simulink model "Grid_Following_Inverters"  (R2024b)
settings: Solver=VariableStepAuto  StartTime=0.0  StopTime=1  RelTol=1e-3
InitFcn:
  | addpath(genpath(fullfile(fileparts(fileparts(fileparts(get_param(bdroot,'FileName')))),'code','functions')));initialize_equipment_model_from_callback(bdroot);
undefined symbols (not defined in the file): Cf, CL, Delta_Iq_LVRT_max, f, I_base, I_limit, I_N, Id_ref_manual, Iq_ref_manual, K_q_LVRT, L1, L2, Lg, Manual_Current_Ref, PLL, PQ, R_C, R_L1, R_L2, Rg, V_base_phase, V_in, V_LVRT_max, V_LVRT_min, Vg
libraries: spsabctodq0Lib x4, spsControlledVoltageSourceLib x3, spsCurrentMeasurementLib x3, spsThreePhaseSeriesRLCBranchLib x3, spsVoltageMeasurementLib x3, spsThreePhaseVIMeasurementLib x2, slpidlib x2, spsGroundLib x1, spsPLL3phLib x1, spsdq0toabcLib x1, spsThreePhaseBreakerLib x1, spsThreePhaseSourceLib x1
settings Model: Creator=ANYE  LastModifiedBy=AnYe
settings SolverCC: ZeroCrossAlgorithm=Adaptive
settings OptimizationCC: ReuseModelBlockBuffer=off
settings DebuggingCC: AlgebraicLoopMsg=none  IgnoredZcDiagnostic=none
settings RTWCC: GPUComputeCapability=3.5

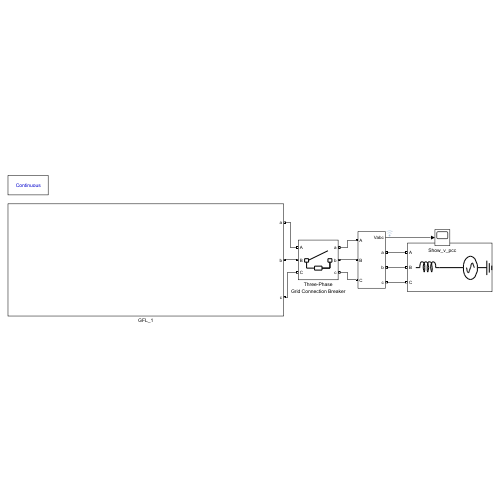
[thumbnail: Simulink's stored preview of the top-level diagram]
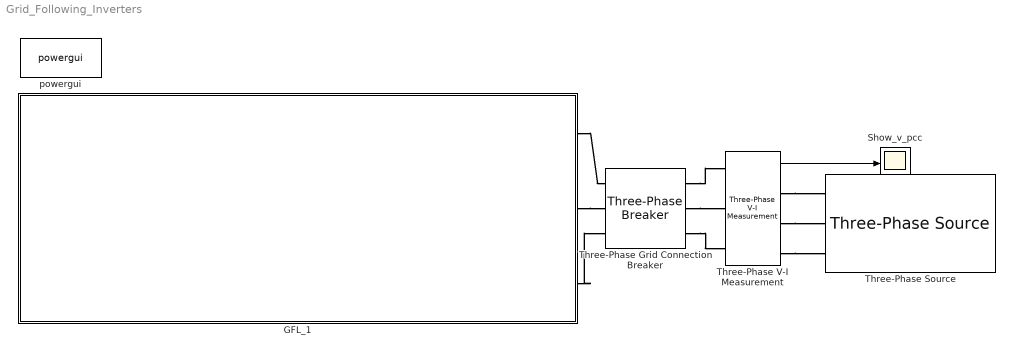
== system Grid_Following_Inverters ==
  GFL_1 : Subsystem
  Show_v_pcc : Scope
  Three-Phase Grid Connection Breaker : spsThreePhaseBreakerLib/Three-Phase Breaker  InitialState=open  SwitchA=on  SwitchB=on  SwitchC=on  SwitchTimes=t_close  External=off  BreakerResistance=0.01  SnubberResistance=1e6  SnubberCapacitance=inf  Measurements=None
  Three-Phase V-I Measurement : spsThreePhaseVIMeasurementLib/Three-Phase V-I Measurement  VoltageMeasurement=phase-to-ground  SetLabelV=off  LabelV=Vabc  Vpu=off  VpuLL=off  CurrentMeasurement=no  SetLabelI=off  LabelI=Iabc  Ipu=off  Pbase=100e6  Vbase=500e3  OutputType=Complex  PhasorSimulation=off  PSBequivalent=0
  Three-Phase Source : spsThreePhaseSourceLib/Three-Phase Source  InternalConnection=Yg  VoltagePhases=off  Voltage=Vg  PhaseAngle=0  Voltage_phases=[25e3 25e3 25e3]/sqrt(3)  PhaseAngles_phases=[0 -120 +120]  Frequency=f  NonIdealSource=on  SpecifyImpedance=off  Resistance=Rg  Inductance=Lg  ShortCircuitLevel=100e6  BaseVoltage=220  XRratio=7  BusType=swing  Pref=10e3  Qref=0  Prefabc=[10e3, 10e3, 10e3]  Qrefabc=[0, 0, 0]  Qmin=-inf  Qmax=inf
      link override Goto: TagVisibility=global
  powergui : spspowerguiLib/powergui  Priority=1  SimulationMode=Continuous  SampleTime=50e-6  frequency=f  Iterations=50  frequencyindice=50  Pbase=100e6  ErrMax=1e-4  UnitsV=kV  UnitsW=MW  buscounter=0  FunctionMessages=off  echomessages=off  EnableUseOfTLC=off  CurrentSourceSwitches=off  DisableSnubberDevices=off  DisableRonSwitches=off  DisableVfSwitches=off  DisplayEquations=off  AutomaticDiscreteSolvers=off  SolverType=Tustin/Backward Euler (TBE)  Interpol=off  ExternalGateDelay=off  methode=off  Ts=100  x0status=blocks  SPID=on  SwTol=0  HookPort=off  NonlinearTolerance=1e-4  nMaxIteration=100  ContinueOnMaxIteration=off  RestoreLinks=warning  ResistiveCurrentMeasurement=off  Frange=[0:2:500]  Ylog=off  Xlog=on  ShowGrid=off  save=off  variable=ZData  structure=0  ZoomFFT=off  StartTime=0.0  cycles=1  DisplayStyle=1  fundamental=f  FreqAxis=off  MaxFrequency=1000  frequencyindicesteady=1  RmsSteady=1  display=off
  wires:
  Three-Phase V-I Measurement/1 -> Show_v_pcc/1
  connections:
  Three-Phase V-I Measurement/RConn1 -- Three-Phase Source/RConn1
  Three-Phase V-I Measurement/RConn2 -- Three-Phase Source/RConn2
  Three-Phase V-I Measurement/RConn3 -- Three-Phase Source/RConn3
  GFL_1/RConn1 -- Three-Phase Grid Connection Breaker/LConn1
  Three-Phase Grid Connection Breaker/RConn1 -- Three-Phase V-I Measurement/LConn1
  GFL_1/RConn2 -- Three-Phase Grid Connection Breaker/LConn2
  Three-Phase Grid Connection Breaker/RConn2 -- Three-Phase V-I Measurement/LConn2
  GFL_1/RConn3 -- Three-Phase Grid Connection Breaker/LConn3
  Three-Phase Grid Connection Breaker/RConn3 -- Three-Phase V-I Measurement/LConn3

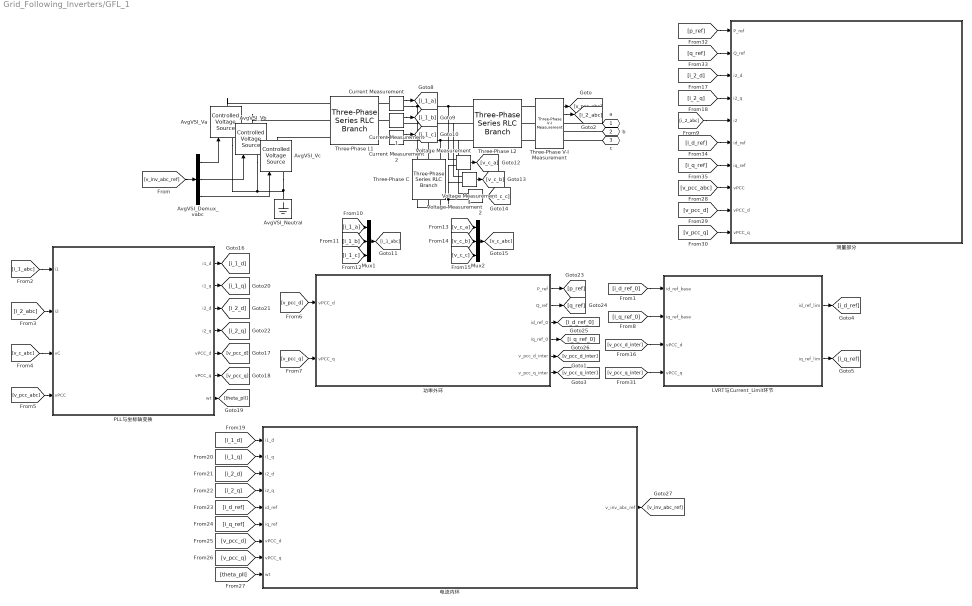
== system Grid_Following_Inverters/GFL_1 ==
  AvgVSI_Demux_vabc : Demux  Outputs=3
  AvgVSI_Neutral : spsGroundLib/Ground  LConnTagsString=a
  AvgVSI_Va : spsControlledVoltageSourceLib/Controlled Voltage Source  Initialize=on  Source_Type=AC  Amplitude=0  Phase=0  Frequency=0  Measurements=None
  AvgVSI_Vb : spsControlledVoltageSourceLib/Controlled Voltage Source  Initialize=on  Source_Type=AC  Amplitude=0  Phase=0  Frequency=0  Measurements=None
  AvgVSI_Vc : spsControlledVoltageSourceLib/Controlled Voltage Source  Initialize=on  Source_Type=AC  Amplitude=0  Phase=0  Frequency=0  Measurements=None
  Current Measurement : spsCurrentMeasurementLib/Current Measurement  PhasorSimulation=off  OutputType=Complex  PSBequivalent=0
  Current Measurement1 : spsCurrentMeasurementLib/Current Measurement  PhasorSimulation=off  OutputType=Complex  PSBequivalent=0
  Current Measurement2 : spsCurrentMeasurementLib/Current Measurement  PhasorSimulation=off  OutputType=Complex  PSBequivalent=0
  LVRT与Current_Limit环节 : Subsystem
  Mux1 : Mux  Inputs=3
  Mux2 : Mux  Inputs=3
  PLL与坐标轴变换 : Subsystem
  Three-Phase C : spsThreePhaseSeriesRLCBranchLib/Three-Phase Series RLC Branch  LConnTagsString=A|B|C  RConnTagsString=A|B|C  BranchType=RC  Resistance=R_C  Inductance=1e-6  Capacitance=Cf  Measurements=None
  Three-Phase L1 : spsThreePhaseSeriesRLCBranchLib/Three-Phase Series RLC Branch  LConnTagsString=A|B|C  RConnTagsString=A|B|C  BranchType=RL  Resistance=R_L1  Inductance=L1  Capacitance=1e-6  Measurements=None
  Three-Phase L2 : spsThreePhaseSeriesRLCBranchLib/Three-Phase Series RLC Branch  LConnTagsString=A|B|C  RConnTagsString=A|B|C  BranchType=RL  Resistance=R_L2  Inductance=L2  Capacitance=1e-6  Measurements=None
  Three-Phase V-I Measurement : spsThreePhaseVIMeasurementLib/Three-Phase V-I Measurement  VoltageMeasurement=phase-to-ground  SetLabelV=off  LabelV=Vabc  Vpu=off  VpuLL=off  CurrentMeasurement=yes  SetLabelI=off  LabelI=Iabc  Ipu=off  Pbase=100e6  Vbase=500e3  OutputType=Complex  PhasorSimulation=off  PSBequivalent=0
  Voltage Measurement : spsVoltageMeasurementLib/Voltage Measurement  PhasorSimulation=off  OutputType=Complex  PSBequivalent=0
  Voltage Measurement1 : spsVoltageMeasurementLib/Voltage Measurement  PhasorSimulation=off  OutputType=Complex  PSBequivalent=0
  Voltage Measurement2 : spsVoltageMeasurementLib/Voltage Measurement  PhasorSimulation=off  OutputType=Complex  PSBequivalent=0
  功率外环 : Subsystem
  测量部分 : Subsystem
  电流内环 : Subsystem
  a : PMIOPort  Side=Right
  b : PMIOPort  Port=2  Side=Right
  c : PMIOPort  Port=3  Side=Right
  wires:
  Three-Phase V-I Measurement/1 -> [v_pcc_abc]
  Current Measurement/1 -> [i_1_a]
  Current Measurement1/1 -> [i_1_b]
  Current Measurement2/1 -> [i_1_c]
  Voltage Measurement1/1 -> [v_c_b]
  Three-Phase V-I Measurement/2 -> [i_2_abc]
  Voltage Measurement2/1 -> [v_c_c]
  Voltage Measurement/1 -> [v_c_a]
  Mux2/1 -> [v_c_abc]
  Mux1/1 -> [i_1_abc]
  [i_1_c] -> Mux1/3
  [v_c_c] -> Mux2/3
  [v_c_b] -> Mux2/2
  [v_c_a] -> Mux2/1
  [i_1_a] -> Mux1/1
  [i_1_b] -> Mux1/2
  PLL与坐标轴变换/6(vPCC_q) -> [v_pcc_q]
  PLL与坐标轴变换/3(i2_d) -> [i_2_d]
  [v_pcc_abc] -> PLL与坐标轴变换/4(vPCC)
  PLL与坐标轴变换/5(vPCC_d) -> [v_pcc_d]
  [v_c_abc] -> PLL与坐标轴变换/3(vC)
  PLL与坐标轴变换/2(i1_q) -> [i_1_q]
  PLL与坐标轴变换/1(i1_d) -> [i_1_d]
  PLL与坐标轴变换/7(wt) -> [theta_pll]
  PLL与坐标轴变换/4(i2_q) -> [i_2_q]
  [i_1_abc] -> PLL与坐标轴变换/1(i1)
  [i_2_abc] -> PLL与坐标轴变换/2(i2)
  功率外环/3(id_ref_0) -> [i_d_ref_0]
  [v_pcc_q] -> 功率外环/2(vPCC_q)
  功率外环/1(P_ref) -> [p_ref]
  功率外环/2(Q_ref) -> [q_ref]
  功率外环/4(iq_ref_0) -> [i_q_ref_0]
  [v_pcc_d] -> 功率外环/1(vPCC_d)
  [i_d_ref] -> 电流内环/5(id_ref)
  [i_q_ref] -> 电流内环/6(iq_ref)
  [v_pcc_d] -> 电流内环/7(vPCC_d)
  [i_1_q] -> 电流内环/2(i1_q)
  [v_pcc_q] -> 电流内环/8(vPCC_q)
  [i_2_d] -> 电流内环/3(i2_d)
  [i_1_d] -> 电流内环/1(i1_d)
  [i_2_q] -> 电流内环/4(i2_q)
  [theta_pll] -> 电流内环/9(wt)
  [i_2_d] -> 测量部分/3(i2_d)
  [i_d_ref] -> 测量部分/6(id_ref)
  [v_pcc_q] -> 测量部分/10(vPCC_q)
  [i_2_q] -> 测量部分/4(i2_q)
  [q_ref] -> 测量部分/2(Q_ref)
  [v_pcc_d] -> 测量部分/9(vPCC_d)
  [p_ref] -> 测量部分/1(P_ref)
  [i_q_ref] -> 测量部分/7(iq_ref)
  [i_2_abc] -> 测量部分/5(i2)
  [v_pcc_abc] -> 测量部分/8(vPCC)
  [v_inv_abc_ref] -> AvgVSI_Demux_vabc/1
  AvgVSI_Demux_vabc/1 -> AvgVSI_Va/1
  AvgVSI_Demux_vabc/2 -> AvgVSI_Vb/1
  AvgVSI_Demux_vabc/3 -> AvgVSI_Vc/1
  电流内环/1(v_inv_abc_ref) -> [v_inv_abc_ref]
  [i_q_ref_0] -> LVRT与Current_Limit环节/2(iq_ref_base)
  [i_d_ref_0] -> LVRT与Current_Limit环节/1(id_ref_base)
  功率外环/5(v_pcc_d_inter) -> [v_pcc_d_inter]
  功率外环/6(v_pcc_q_inter) -> [v_pcc_q_inter]
  [v_pcc_d_inter] -> LVRT与Current_Limit环节/3(vPCC_d)
  [v_pcc_q_inter] -> LVRT与Current_Limit环节/4(vPCC_q)
  LVRT与Current_Limit环节/1(id_ref_lim) -> [i_d_ref]
  LVRT与Current_Limit环节/2(iq_ref_lim) -> [i_q_ref]
  connections:
  Current Measurement1/LConn1 -- Three-Phase L1/RConn2
  a/RConn1 -- Three-Phase V-I Measurement/RConn1
  Three-Phase C/RConn1 -- Voltage Measurement2/LConn2 -- Voltage Measurement1/LConn2 -- Voltage Measurement/LConn2 -- Three-Phase C/RConn3 -- Three-Phase C/RConn2
  Three-Phase C/LConn2 -- Three-Phase L2/LConn2 -- Voltage Measurement1/LConn1 -- Current Measurement1/RConn1
  Three-Phase C/LConn3 -- Three-Phase L2/LConn3 -- Voltage Measurement2/LConn1 -- Current Measurement2/RConn1
  Three-Phase V-I Measurement/LConn2 -- Three-Phase L2/RConn2
  Three-Phase C/LConn1 -- Current Measurement/RConn1 -- Three-Phase L2/LConn1 -- Voltage Measurement/LConn1
  Three-Phase L1/RConn3 -- Current Measurement2/LConn1
  Current Measurement/LConn1 -- Three-Phase L1/RConn1
  Three-Phase V-I Measurement/LConn3 -- Three-Phase L2/RConn3
  b/RConn1 -- Three-Phase V-I Measurement/RConn2
  Three-Phase V-I Measurement/LConn1 -- Three-Phase L2/RConn1
  c/RConn1 -- Three-Phase V-I Measurement/RConn3
  AvgVSI_Vb/RConn1 -- Three-Phase L1/LConn2
  AvgVSI_Va/RConn1 -- Three-Phase L1/LConn1
  Three-Phase L1/LConn3 -- AvgVSI_Vc/RConn1
  AvgVSI_Va/LConn1 -- AvgVSI_Vc/LConn1 -- AvgVSI_Neutral/LConn1 -- AvgVSI_Vb/LConn1

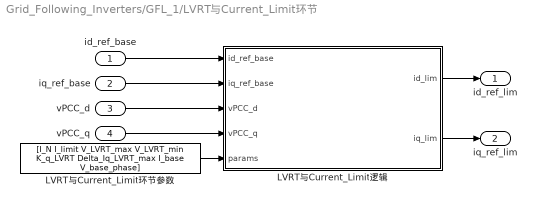
== system Grid_Following_Inverters/GFL_1/LVRT与Current_Limit环节 ==
  id_ref_base : Inport
  iq_ref_base : Inport  Port=2
  vPCC_d : Inport  Port=3
  vPCC_q : Inport  Port=4
  LVRT与Current_Limit环节参数 : Constant  Value=[I_N I_limit V_LVRT_max V_LVRT_min K_q_LVRT Delta_Iq_LVRT_max I_base V_base_phase]
  LVRT与Current_Limit逻辑 : MATLAB Function  TreatAsAtomicUnit=on
  id_ref_lim : Outport
  iq_ref_lim : Outport  Port=2
  wires:
  id_ref_base/1 -> LVRT与Current_Limit逻辑/1(id_ref_base)
  iq_ref_base/1 -> LVRT与Current_Limit逻辑/2(iq_ref_base)
  vPCC_d/1 -> LVRT与Current_Limit逻辑/3(vPCC_d)
  vPCC_q/1 -> LVRT与Current_Limit逻辑/4(vPCC_q)
  LVRT与Current_Limit环节参数/1 -> LVRT与Current_Limit逻辑/5(params)
  LVRT与Current_Limit逻辑/1(id_lim) -> id_ref_lim/1
  LVRT与Current_Limit逻辑/2(iq_lim) -> iq_ref_lim/1

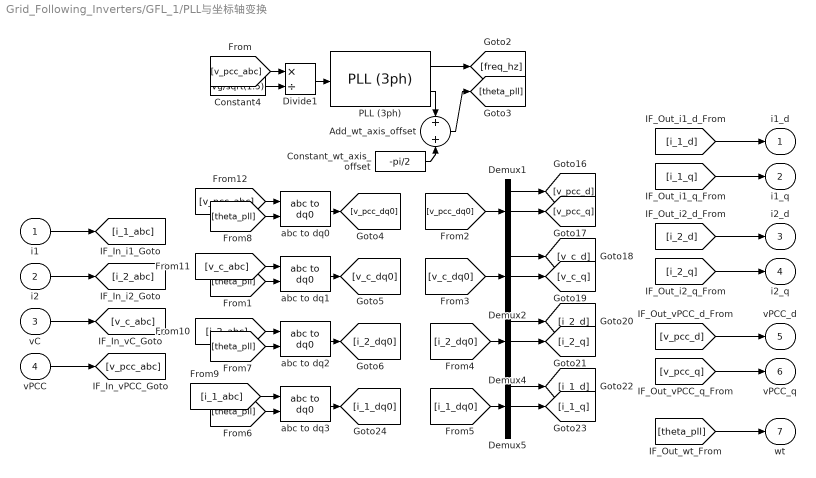
== system Grid_Following_Inverters/GFL_1/PLL与坐标轴变换 ==
  i1 : Inport
  i2 : Inport  Port=2
  vC : Inport  Port=3
  vPCC : Inport  Port=4
  Add_wt_axis_offset : Sum
  Constant4 : Constant  Value=Vg/sqrt(1.5)
  Constant_wt_axis_offset : Constant  Value=-pi/2
  Demux{1..2,4..5} (4 alike) : Demux  Outputs=3
  Divide1 : Product  Inputs=*/
  PLL (3ph) : spsPLL3phLib/PLL (3ph)  Fmin=45  Par_Init=[0, 50]  ParK=[PLL.Kp, PLL.Ki, PLL.Kd]  TcD=1e-4  MaxRateChangeFreq=12  FilterCutOffFreq=25  Ts=0  AGC=on
  abc to dq{0..3} (4 alike) : spsabctodq0Lib/abc to dq0  Alignment=Aligned with phase A axis
  i1_d : Outport
  i1_q : Outport  Port=2
  i2_d : Outport  Port=3
  i2_q : Outport  Port=4
  vPCC_d : Outport  Port=5
  vPCC_q : Outport  Port=6
  wt : Outport  Port=7
  wires:
  PLL (3ph)/1 -> [freq_hz]
  abc to dq0/1 -> [v_pcc_dq0]
  Demux1/1 -> [v_pcc_d]
  Add_wt_axis_offset/1 -> [theta_pll]
  [v_c_dq0] -> Demux2/1
  Demux4/2 -> [i_2_q]
  PLL (3ph)/2 -> Add_wt_axis_offset/1
  Demux2/2 -> [v_c_q]
  [theta_pll] -> abc to dq2/2
  Demux1/2 -> [v_pcc_q]
  [v_pcc_dq0] -> Demux1/1
  Demux2/1 -> [v_c_d]
  [theta_pll] -> abc to dq3/2
  Demux4/1 -> [i_2_d]
  [v_pcc_abc] -> abc to dq0/1
  abc to dq3/1 -> [i_1_dq0]
  Divide1/1 -> PLL (3ph)/1
  [i_1_abc] -> abc to dq3/1
  [theta_pll] -> abc to dq0/2
  [i_2_abc] -> abc to dq2/1
  [theta_pll] -> abc to dq1/2
  [i_2_dq0] -> Demux4/1
  Demux5/1 -> [i_1_d]
  [v_c_abc] -> abc to dq1/1
  [i_1_dq0] -> Demux5/1
  Constant4/1 -> Divide1/2
  abc to dq2/1 -> [i_2_dq0]
  [v_pcc_abc] -> Divide1/1
  abc to dq1/1 -> [v_c_dq0]
  Constant_wt_axis_offset/1 -> Add_wt_axis_offset/2
  Demux5/2 -> [i_1_q]
  i1/1 -> [i_1_abc]
  [i_1_d] -> i1_d/1
  [i_1_q] -> i1_q/1
  i2/1 -> [i_2_abc]
  [i_2_d] -> i2_d/1
  [i_2_q] -> i2_q/1
  vC/1 -> [v_c_abc]
  vPCC/1 -> [v_pcc_abc]
  [v_pcc_d] -> vPCC_d/1
  [v_pcc_q] -> vPCC_q/1
  [theta_pll] -> wt/1

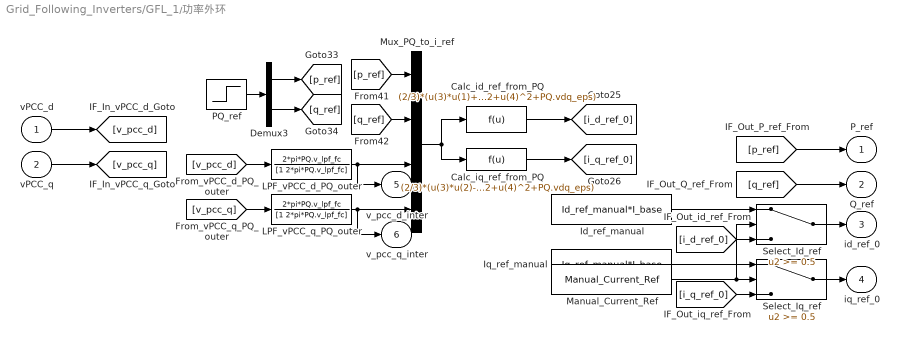
== system Grid_Following_Inverters/GFL_1/功率外环 ==
  vPCC_d : Inport
  vPCC_q : Inport  Port=2
  Calc_id_ref_from_PQ : Fcn  Expr=(2/3)*(u(3)*u(1)+u(4)*u(2))/(u(3)^2+u(4)^2+PQ.vdq_eps)
  Calc_iq_ref_from_PQ : Fcn  Expr=(2/3)*(u(3)*u(2)-u(4)*u(1))/(u(3)^2+u(4)^2+PQ.vdq_eps)
  Demux3 : Demux  Outputs=2
  Id_ref_manual : Constant  Value=Id_ref_manual*I_base
  Iq_ref_manual : Constant  Value=Iq_ref_manual*I_base
  LPF_vPCC_d_PQ_outer : TransferFcn  Numerator=2*pi*PQ.v_lpf_fc  Denominator=[1 2*pi*PQ.v_lpf_fc]
  LPF_vPCC_q_PQ_outer : TransferFcn  Numerator=2*pi*PQ.v_lpf_fc  Denominator=[1 2*pi*PQ.v_lpf_fc]
  Manual_Current_Ref : Constant  Value=Manual_Current_Ref
  Mux_PQ_to_i_ref : Mux
  PQ_ref : Step  Time=[PQ.step_time_P PQ.step_time_Q]  After=[PQ.Pref,PQ.Qref]  SampleTime=0
  Select_Id_ref : Switch  Threshold=0.5  SaturateOnIntegerOverflow=off  InputSameDT=off
  Select_Iq_ref : Switch  Threshold=0.5  SaturateOnIntegerOverflow=off  InputSameDT=off
  P_ref : Outport
  Q_ref : Outport  Port=2
  id_ref_0 : Outport  Port=3
  iq_ref_0 : Outport  Port=4
  v_pcc_d_inter : Outport  Port=5
  v_pcc_q_inter : Outport  Port=6
  wires:
  [v_pcc_q] -> LPF_vPCC_q_PQ_outer/1
  [p_ref] -> Mux_PQ_to_i_ref/1
  [q_ref] -> Mux_PQ_to_i_ref/2
  Demux3/1 -> [p_ref]
  LPF_vPCC_d_PQ_outer/1 -> Mux_PQ_to_i_ref/3, v_pcc_d_inter/1
  Mux_PQ_to_i_ref/1 -> Calc_id_ref_from_PQ/1, Calc_iq_ref_from_PQ/1
  [v_pcc_d] -> LPF_vPCC_d_PQ_outer/1
  LPF_vPCC_q_PQ_outer/1 -> v_pcc_q_inter/1, Mux_PQ_to_i_ref/4
  PQ_ref/1 -> Demux3/1
  Demux3/2 -> [q_ref]
  [p_ref] -> P_ref/1
  [q_ref] -> Q_ref/1
  vPCC_q/1 -> [v_pcc_q]
  vPCC_d/1 -> [v_pcc_d]
  Calc_id_ref_from_PQ/1 -> [i_d_ref_0]
  Calc_iq_ref_from_PQ/1 -> [i_q_ref_0]
  Id_ref_manual/1 -> Select_Id_ref/1
  Manual_Current_Ref/1 -> Select_Id_ref/2, Select_Iq_ref/2
  [i_d_ref_0] -> Select_Id_ref/3
  Select_Id_ref/1 -> id_ref_0/1
  Iq_ref_manual/1 -> Select_Iq_ref/1
  [i_q_ref_0] -> Select_Iq_ref/3
  Select_Iq_ref/1 -> iq_ref_0/1

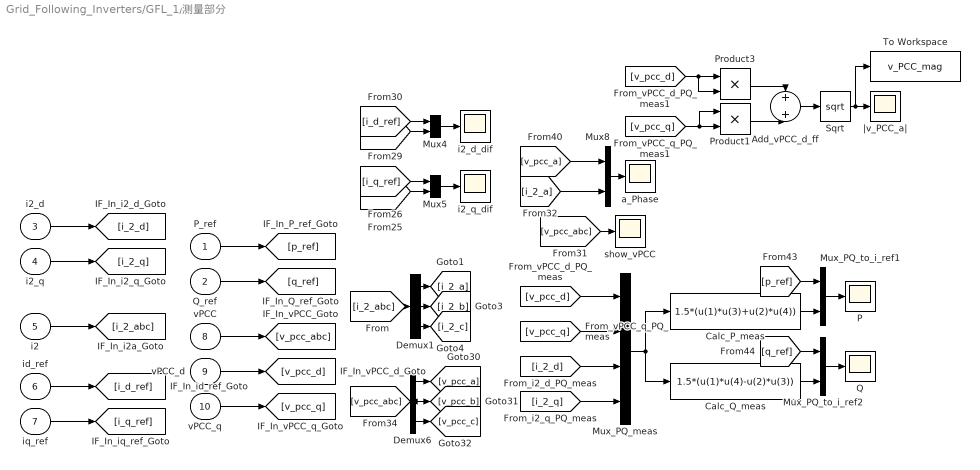
== system Grid_Following_Inverters/GFL_1/测量部分 ==
  P_ref : Inport
  Q_ref : Inport  Port=2
  i2_d : Inport  Port=3
  i2_q : Inport  Port=4
  i2 : Inport  Port=5
  id_ref : Inport  Port=6
  iq_ref : Inport  Port=7
  vPCC : Inport  Port=8
  vPCC_d : Inport  Port=9
  vPCC_q : Inport  Port=10
  Add_vPCC_d_ff : Sum
  Calc_P_meas : Fcn  Expr=1.5*(u(1)*u(3)+u(2)*u(4))
  Calc_Q_meas : Fcn  Expr=1.5*(u(1)*u(4)-u(2)*u(3))
  Demux1 : Demux  Outputs=3
  Demux6 : Demux  Outputs=3
  Mux4 : Mux  Inputs=2
  Mux5 : Mux  Inputs=2
  Mux8 : Mux  Inputs=2
  Mux_PQ_meas : Mux
  Mux_PQ_to_i_ref1 : Mux  Inputs=2
  Mux_PQ_to_i_ref2 : Mux  Inputs=2
  P : Scope
  Product1 : Product
  Product3 : Product
  Q : Scope
  Sqrt : Sqrt
  To Workspace : ToWorkspace  VariableName=v_PCC_mag  SaveFormat=Timeseries  SampleTime=-1
  a_Phase : Scope
  i2_d_dif : Scope
  i2_q_dif : Scope
  show_vPCC : Scope
  |v_PCC_a| : Scope
  wires:
  [q_ref] -> Mux_PQ_to_i_ref2/1
  [v_pcc_d] -> Mux_PQ_meas/1
  [i_2_d] -> Mux_PQ_meas/3
  [i_2_q] -> Mux_PQ_meas/4
  Mux4/1 -> i2_d_dif/1
  [v_pcc_a] -> Mux8/1
  [v_pcc_abc] -> Demux6/1
  [i_d_ref] -> Mux4/1
  [v_pcc_abc] -> show_vPCC/1
  [i_2_d] -> Mux4/2
  Demux6/1 -> [v_pcc_a]
  [i_2_a] -> Mux8/2
  Mux_PQ_to_i_ref2/1 -> Q/1
  [i_2_q] -> Mux5/2
  [p_ref] -> Mux_PQ_to_i_ref1/1
  [i_q_ref] -> Mux5/1
  Mux_PQ_meas/1 -> Calc_P_meas/1, Calc_Q_meas/1
  Demux6/2 -> [v_pcc_b]
  Calc_Q_meas/1 -> Mux_PQ_to_i_ref2/2
  Mux5/1 -> i2_q_dif/1
  [v_pcc_q] -> Mux_PQ_meas/2
  Mux8/1 -> a_Phase/1
  Mux_PQ_to_i_ref1/1 -> P/1
  Calc_P_meas/1 -> Mux_PQ_to_i_ref1/2
  Demux6/3 -> [v_pcc_c]
  P_ref/1 -> [p_ref]
  Q_ref/1 -> [q_ref]
  i2_d/1 -> [i_2_d]
  i2_q/1 -> [i_2_q]
  i2/1 -> [i_2_abc]
  id_ref/1 -> [i_d_ref]
  iq_ref/1 -> [i_q_ref]
  vPCC/1 -> [v_pcc_abc]
  vPCC_d/1 -> [v_pcc_d]
  vPCC_q/1 -> [v_pcc_q]
  Demux1/1 -> [i_2_a]
  [i_2_abc] -> Demux1/1
  Demux1/3 -> [i_2_c]
  Demux1/2 -> [i_2_b]
  [v_pcc_d] -> Product3/2, Product3/1
  [v_pcc_q] -> Product1/1, Product1/2
  Add_vPCC_d_ff/1 -> Sqrt/1
  Product3/1 -> Add_vPCC_d_ff/1
  Product1/1 -> Add_vPCC_d_ff/2
  Sqrt/1 -> To Workspace/1, |v_PCC_a|/1

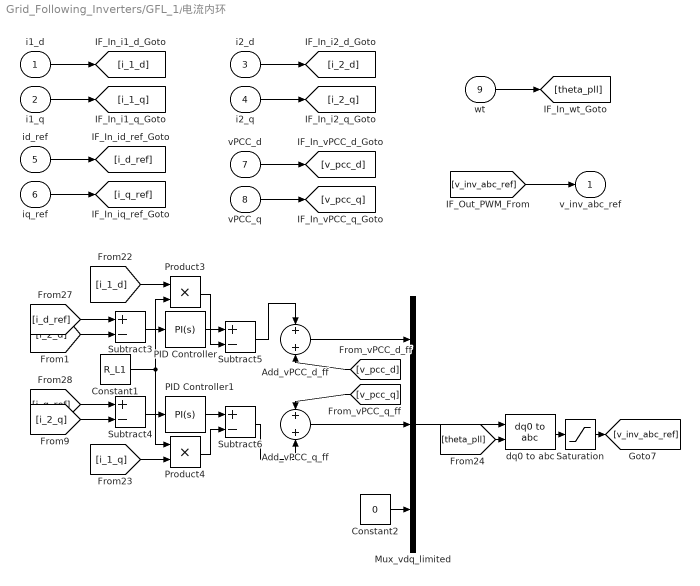
== system Grid_Following_Inverters/GFL_1/电流内环 ==
  i1_d : Inport
  i1_q : Inport  Port=2
  i2_d : Inport  Port=3
  i2_q : Inport  Port=4
  id_ref : Inport  Port=5
  iq_ref : Inport  Port=6
  vPCC_d : Inport  Port=7
  vPCC_q : Inport  Port=8
  wt : Inport  Port=9
  Add_vPCC_d_ff : Sum
  Add_vPCC_q_ff : Sum
  Constant1 : Constant  Value=R_L1
  Constant2 : Constant  Value=0
  Mux_vdq_limited : Mux  Inputs=3
  PID Controller : slpidlib/PID Controller  Controller=PI  Form=Parallel  TimeDomain=Continuous-time  UseExternalTs=off  SampleTime=-1  IntegratorMethod=Forward Euler  FilterMethod=Forward Euler  ControllerParametersSource=internal  P=CL.Kp  I=CL.Ki  UseKiTs=off  D=0  UseExternalDerivativeSource=off  N=100  UseFilter=on  TunerSelectOption=Transfer Function Based (PID Tuner App)  InitialConditionSource=internal  InitialConditionForIntegrator=0  InitialConditionForFilter=0  DifferentiatorICPrevScaledInput=0  ExternalReset=none  TrackingMode=off  Kt=1  LimitOutput=off  SatLimitsSource=internal  UpperSaturationLimit=inf  LowerSaturationLimit=-inf  LinearizeAsGain=on  AntiWindupMode=none  Kb=1  LimitIntegrator=off  UpperIntegratorSaturationLimit=inf  LowerIntegratorSaturationLimit=-inf  POutMin=[]  POutMax=[]  IOutMin=[]  IOutMax=[]  DOutMin=[]  DOutMax=[]  NOutMin=[]  NOutMax=[]  SumOutMin=[]  SumOutMax=[]  SaturationOutMin=[]  SaturationOutMax=[]  PParamMin=[]  PParamMax=[]  IParamMin=[]  IParamMax=[]  DParamMin=[]  DParamMax=[]  NParamMin=[]  NParamMax=[]  KbParamMin=[]  KbParamMax=[]  KtParamMin=[]  KtParamMax=[]  KbOutMin=[]  KbOutMax=[]  KtOutMin=[]  KtOutMax=[]  IntegratorOutMin=[]  IntegratorOutMax=[]  FilterOutMin=[]  FilterOutMax=[]  SumI1OutMin=[]  SumI1OutMax=[]  SumI2OutMin=[]  SumI2OutMax=[]  SumI3OutMin=[]  SumI3OutMax=[]  SumI4OutMin=[]  SumI4OutMax=[]  SumDOutMin=[]  SumDOutMax=[]  DifferentiatorOutMin=[]  DifferentiatorOutMax=[]  FilterDiffOutCoefMin=[]  FilterDiffOutCoefMax=[]  ReciprocalOutMin=[]  ReciprocalOutMax=[]  SumDenOutMin=[]  SumDenOutMax=[]  SumNumOutMin=[]  SumNumOutMax=[]  DivideOutMin=[]  DivideOutMax=[]  UdiffTsProdOutMin=[]  UdiffTsProdOutMax=[]  NTsProdOutMin=[]  NTsProdOutMax=[]  UintegralTsProdOutMin=[]  UintegralTsProdOutMax=[]  UngainTsProdOutMin=[]  UngainTsProdOutMax=[]  ClampingZeroOutDataTypeStr=Inherit: Inherit via back propagation  ClampingZeroOutMin=[]  ClampingZeroOutMax=[]  FilterDenConstantOutDataTypeStr=Inherit: Inherit via back propagation  FilterDenConstantOutMin=[]  FilterDenConstantOutMax=[]  PCopyOutDataTypeStr=Inherit: Inherit via back propagation  PCopyOutMin=[]  PCopyOutMax=[]  NCopyOutDataTypeStr=Inherit: Inherit via back propagation  NCopyOutMin=[]  NCopyOutMax=[]  IntegratorContinuousStateAttributes=''  IntegratorStateMustResolveToSignalObject=off  IntegratorRTWStateStorageClass=Auto  FilterContinuousStateAttributes=''  FilterStateMustResolveToSignalObject=off  FilterRTWStateStorageClass=Auto  ParallelPVariant=InternalParameters  IdealPVariant=Disabled  IVariant=InternalParameters  DVariant=Disabled  IntegratorVariant=Continuous  SatVariant=Disabled  AWVariant=Passthrough  PCopyVariant=Disabled  TRVariant=Disabled  FdbkBlocksVariant=Forward  IdealPFdbkVariant=Disabled  SatFdbkVariant=Disabled  DerivativeFilterVariant=Disabled  NVariant=Disabled  NCopyVariant=Disabled_SignalSpec  FilterICVariant=Disabled  IntegratorICVariant=InternalICs  ExternalResetVariant=Disabled  TRSumVariant=Passthrough  SumFdbkVariant=Disabled  SumVariant=Sum_PI  TsampFilterVariant=InternalTs  TsampNgainVariant=Passthrough  TsampIntegralVariant=Disabled_SignalSpec  ExternalSaturationOutDataTypeStr=Inherit: Same as second input  DerivativeSourceVariant=Disabled  PreIntVariant=InternalPreInt
  PID Controller1 : slpidlib/PID Controller  Controller=PI  Form=Parallel  TimeDomain=Continuous-time  UseExternalTs=off  SampleTime=-1  IntegratorMethod=Forward Euler  FilterMethod=Forward Euler  ControllerParametersSource=internal  P=CL.Kp  I=CL.Ki  UseKiTs=off  D=0  UseExternalDerivativeSource=off  N=100  UseFilter=on  TunerSelectOption=Transfer Function Based (PID Tuner App)  InitialConditionSource=internal  InitialConditionForIntegrator=0  InitialConditionForFilter=0  DifferentiatorICPrevScaledInput=0  ExternalReset=none  TrackingMode=off  Kt=1  LimitOutput=off  SatLimitsSource=internal  UpperSaturationLimit=inf  LowerSaturationLimit=-inf  LinearizeAsGain=on  AntiWindupMode=none  Kb=1  LimitIntegrator=off  UpperIntegratorSaturationLimit=inf  LowerIntegratorSaturationLimit=-inf  POutMin=[]  POutMax=[]  IOutMin=[]  IOutMax=[]  DOutMin=[]  DOutMax=[]  NOutMin=[]  NOutMax=[]  SumOutMin=[]  SumOutMax=[]  SaturationOutMin=[]  SaturationOutMax=[]  PParamMin=[]  PParamMax=[]  IParamMin=[]  IParamMax=[]  DParamMin=[]  DParamMax=[]  NParamMin=[]  NParamMax=[]  KbParamMin=[]  KbParamMax=[]  KtParamMin=[]  KtParamMax=[]  KbOutMin=[]  KbOutMax=[]  KtOutMin=[]  KtOutMax=[]  IntegratorOutMin=[]  IntegratorOutMax=[]  FilterOutMin=[]  FilterOutMax=[]  SumI1OutMin=[]  SumI1OutMax=[]  SumI2OutMin=[]  SumI2OutMax=[]  SumI3OutMin=[]  SumI3OutMax=[]  SumI4OutMin=[]  SumI4OutMax=[]  SumDOutMin=[]  SumDOutMax=[]  DifferentiatorOutMin=[]  DifferentiatorOutMax=[]  FilterDiffOutCoefMin=[]  FilterDiffOutCoefMax=[]  ReciprocalOutMin=[]  ReciprocalOutMax=[]  SumDenOutMin=[]  SumDenOutMax=[]  SumNumOutMin=[]  SumNumOutMax=[]  DivideOutMin=[]  DivideOutMax=[]  UdiffTsProdOutMin=[]  UdiffTsProdOutMax=[]  NTsProdOutMin=[]  NTsProdOutMax=[]  UintegralTsProdOutMin=[]  UintegralTsProdOutMax=[]  UngainTsProdOutMin=[]  UngainTsProdOutMax=[]  ClampingZeroOutDataTypeStr=Inherit: Inherit via back propagation  ClampingZeroOutMin=[]  ClampingZeroOutMax=[]  FilterDenConstantOutDataTypeStr=Inherit: Inherit via back propagation  FilterDenConstantOutMin=[]  FilterDenConstantOutMax=[]  PCopyOutDataTypeStr=Inherit: Inherit via back propagation  PCopyOutMin=[]  PCopyOutMax=[]  NCopyOutDataTypeStr=Inherit: Inherit via back propagation  NCopyOutMin=[]  NCopyOutMax=[]  IntegratorContinuousStateAttributes=''  IntegratorStateMustResolveToSignalObject=off  IntegratorRTWStateStorageClass=Auto  FilterContinuousStateAttributes=''  FilterStateMustResolveToSignalObject=off  FilterRTWStateStorageClass=Auto  ParallelPVariant=InternalParameters  IdealPVariant=Disabled  IVariant=InternalParameters  DVariant=Disabled  IntegratorVariant=Continuous  SatVariant=Disabled  AWVariant=Passthrough  PCopyVariant=Disabled  TRVariant=Disabled  FdbkBlocksVariant=Forward  IdealPFdbkVariant=Disabled  SatFdbkVariant=Disabled  DerivativeFilterVariant=Disabled  NVariant=Disabled  NCopyVariant=Disabled_SignalSpec  FilterICVariant=Disabled  IntegratorICVariant=InternalICs  ExternalResetVariant=Disabled  TRSumVariant=Passthrough  SumFdbkVariant=Disabled  SumVariant=Sum_PI  TsampFilterVariant=InternalTs  TsampNgainVariant=Passthrough  TsampIntegralVariant=Disabled_SignalSpec  ExternalSaturationOutDataTypeStr=Inherit: Same as second input  DerivativeSourceVariant=Disabled  PreIntVariant=InternalPreInt
  Product3 : Product
  Product4 : Product
  Saturation : Saturate  UpperLimit=+V_in/2  LowerLimit=-V_in/2
  Subtract{3..6} (4 alike) : Sum  Inputs=+-
  dq0 to abc : spsdq0toabcLib/dq0 to abc  Alignment=Aligned with phase A axis
  v_inv_abc_ref : Outport
  wires:
  [i_d_ref] -> Subtract3/1
  Constant1/1 -> Product4/1, Product3/2
  Product4/1 -> Subtract6/2
  PID Controller/1 -> Subtract5/1
  Constant2/1 -> Mux_vdq_limited/3
  [i_1_d] -> Product3/1
  Subtract3/1 -> PID Controller/1
  [i_q_ref] -> Subtract4/1
  [i_2_d] -> Subtract3/2
  Product3/1 -> Subtract5/2
  [i_1_q] -> Product4/2
  Subtract6/1 -> Add_vPCC_q_ff/2
  [i_2_q] -> Subtract4/2
  [theta_pll] -> dq0 to abc/2
  Subtract4/1 -> PID Controller1/1
  Subtract5/1 -> Add_vPCC_d_ff/1
  PID Controller1/1 -> Subtract6/1
  [v_inv_abc_ref] -> v_inv_abc_ref/1
  i1_d/1 -> [i_1_d]
  i1_q/1 -> [i_1_q]
  i2_d/1 -> [i_2_d]
  i2_q/1 -> [i_2_q]
  id_ref/1 -> [i_d_ref]
  iq_ref/1 -> [i_q_ref]
  vPCC_d/1 -> [v_pcc_d]
  vPCC_q/1 -> [v_pcc_q]
  wt/1 -> [theta_pll]
  Mux_vdq_limited/1 -> dq0 to abc/1
  Add_vPCC_d_ff/1 -> Mux_vdq_limited/1
  Add_vPCC_q_ff/1 -> Mux_vdq_limited/2
  [v_pcc_d] -> Add_vPCC_d_ff/2
  [v_pcc_q] -> Add_vPCC_q_ff/1
  dq0 to abc/1 -> Saturation/1
  Saturation/1 -> [v_inv_abc_ref]

== matlab function Grid_Following_Inverters/GFL_1/LVRT与Current_Limit环节/LVRT与Current_Limit逻辑 ==
  data: id_ref_base input; id_lim output; iq_ref_base input; vPCC_d input; vPCC_q input; params input; iq_lim output
function [id_lim, iq_lim] = f(id_ref_base, iq_ref_base, vPCC_d, vPCC_q, params)

I_N          = max(params(1), 0);
I_limit_pu   = max(params(2), 0);
V_LVRT_max   = params(3);
V_LVRT_min   = params(4);
K_q_LVRT     = max(params(5), 0);
Delta_Iq_LVRT_max_pu = max(params(6), 0);
I_base       = max(params(7), eps);
V_base_phase = max(params(8), eps);

v_pcc_pu = sqrt(vPCC_d*vPCC_d+vPCC_q*vPCC_q)/V_base_phase;

I_rated_abs = I_N*I_base;
I_limit_abs = I_limit_pu*I_rated_abs;
Delta_Iq_LVRT_max = Delta_Iq_LVRT_max_pu*I_rated_abs;

if V_LVRT_max > V_LVRT_min
    delta_iq = K_q_LVRT*(V_LVRT_max-v_pcc_pu)*I_rated_abs;
    delta_iq = min(max(delta_iq, 0), Delta_Iq_LVRT_max);
else
    delta_iq = 0;
end

iq_ref = iq_ref_base+delta_iq;
iq_lim = sign(iq_ref)*min(abs(iq_ref), I_limit_abs);

id_available = sqrt(max(I_limit_abs*I_limit_abs - iq_lim*iq_lim, 0));
id_lim       = sign(id_ref_base)*min(abs(id_ref_base), id_available);

end
